simulink library "Parts_Lib"  (R2024a)
settings: Solver=ode45  StartTime=0.0  StopTime=10.0  RelTol=1e-3  EnableMultiTasking=on
undefined symbols (not defined in the file or in its folder): Extr_Data_Ring, X, Y, Z
libraries: sm_lib x44
(part 1 of 2)
Description:
  | Copyright 2015-2024 The MathWorks, Inc.
settings Model: Creator=smiller  LastModifiedBy=smiller
settings SolverCC: AlgebraicLoopSolver=TrustRegion
settings DataIOCC: LimitDataPoints=on  SaveFormat=Array  ReturnWorkspaceOutputs=off
settings OptimizationCC: ReuseModelBlockBuffer=off  LifeSpan=inf
settings DebuggingCC: SolverPrmCheckMsg=warning  UnconnectedInputMsg=warning  UnconnectedOutputMsg=warning  UnconnectedLineMsg=warning  AllowSymbolicDim=off  PregeneratedLibrarySubsystemCodeDiagnostic=none  SFUnexpectedBacktrackingDiag=warning  SFNoUnconditionalDefaultTransitionDiag=warning  SFExecutionAtInitializationDiag=none  ArithmeticOperatorsInVariantConditions=warning
settings HardwareCC: ProdBitPerPointer=32  ProdBitPerSizeT=32  ProdBitPerPtrDiffT=32  ProdLargestAtomicFloat=None  ProdIntDivRoundTo=Undefined  ProdEndianess=Unspecified  ProdWordSize=32  ProdHWDeviceType=32-bit Generic
settings ModelReferenceCC: EnableRefExpFcnMdlSchedulingChecks=on  PropagateSignalLabelsOutOfModel=off
settings SFSimCC: SimUseLocalCustomCode=off  CustomCodeUndefinedFunction=UseInterfaceOnly
settings RTWCC: RTWUseLocalCustomCode=off  GPUComputeCapability=3.5  DLArmComputeVersion=19.05
settings CodeAppCC: StateflowObjectComments=on
settings GRTTargetCC: TargetLangStandard=C89/C90 (ANSI)
settings ConfigComp: CovMetricSettings=dw  CovSaveCumulativeToWorkspaceVar=on  CovSaveSingleToWorkspaceVar=on  CovExternalEMLEnable=off  CovSFcnEnable=off

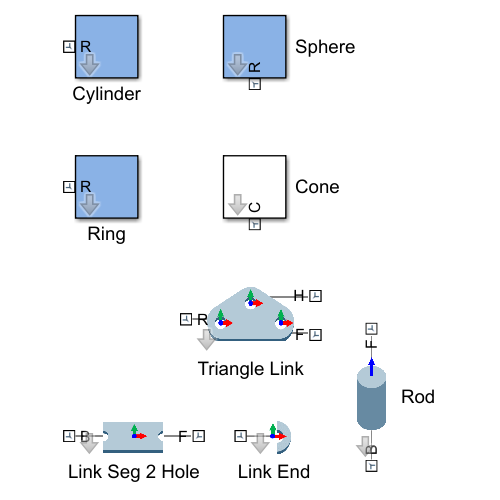
[thumbnail: Simulink's stored preview of the top-level diagram]
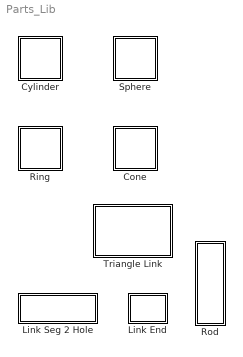
== system Parts_Lib ==
  Cone : Subsystem  mask(Conical Frustrum){cone_or=37.5e-3, cone_ir=30e-3, cone_h=4e-2, cone_theta=60, cone_angle_range=[-180 180], cone_rho=7000, cone_clr=[0.0 0.4 0.6], cone_opc=1, popup_markings=Two, mark_radius_scale=[1.01 1.01], mark_angle_range=2, mark_color=[1 1 1]}
      mask prompts: cone_or "Outer Radius (m):"; cone_ir "Inner Radius (m):"; cone_h "Height (m):"; cone_theta "Angle (deg):"; cone_angle_range "Sweep Angle (min, max angle (deg))"; cone_rho "Density (kg/m^3):"; cone_clr "Color [RGB]:"; cone_opc "Opacity (0-1)"; popup_markings "Show Markings"; mark_radius_scale "Radius scale factor [rad, h] (~1)"; mark_angle_range "Sweep Angle [0-180] (deg)"; mark_color "Color [RGB]"
      mask help:
      | This block models a conical frustrum.
      |
      | The port C corresponds to the frame at one end of the cone whose z-axis points along the cone axis.
      mask init:
      | frcon_xsec = Extr_Data_Frustum_Conical(cone_or, cone_theta, cone_h, cone_ir);
      | mark_xsec = Extr_Data_Frustum_Conical(cone_or*mark_radius_scale(1), cone_theta, cone_h*(1+(mark_radius_scale(2)-1)*2), cone_ir*(2-mark_radius_scale(1)));
      | 
      | mark_xsec(:,2) = mark_xsec(:,2)-cone_h*(mark_radius_scale(2)-1);
      | 
      | mark_1_opc = 0;
      | mark_2_opc = 0;
      | 
      | if(popup_markings == 2)
      |     mark_1_opc = 1;
      | elseif(popup_markings == 3)
      |     mark_1_opc = 1;
      |     mark_2_opc = 1;
      | end
      mask TypeOptions popup_markings: None | One | Two
      mask Callback popup_markings:
      | maskObj = Simulink.Mask.get(gcb);
      | mkc_h = maskObj.getDialogControl('container_markings');
      | if strcmp(get_param(gcb,'popup_markings'),'None')
      |     mkc_h.Visible = 'off';
      | else
      |     mkc_h.Visible = 'on';
      | end
      | clear maskObj mkc_h
      mask DialogControl Control2 Prompt: Plot Profile
      mask DialogControl Control2 Callback:
      | v = get_param(gcb,'MaskWSVariables');
      | getMaskValue = containers.Map({v.Name}',{v.Value}');
      | evalin('base',...
      |     sprintf('Extr_Data_Frustum_Conical(%s,%s,%s,%s,''%s'');',...
      |     num2str(getMaskValue('cone_or')),...
      |     num2str(getMaskValue('cone_theta')),...
      |     num2str(getMaskValue('cone_h')),...
      |     num2str(getMaskValue('cone_ir')),'plot'));
  Cylinder : Subsystem  Tag=CustomStyle  mask(Solid Cylinder with Markings){cyl_radius=0.5, cyl_length=0.2, cyl_density=1000, cyl_color=blue, cyl_opacity=1, cyl_color_custom=[0.7920    0.9900    0.9900], mark_radius=[0.75 0.5], mark_len_factor=1.01, mark_angle=60, mark_color=purple, mark_opacity=1}
      mask prompts: cyl_radius "Radius (m)"; cyl_length "Length (m)"; cyl_density "Density (kg/m^3)"; cyl_color "Color"; cyl_opacity "Opacity (0-1)"; cyl_color_custom "Custom Color (rgb)"; mark_radius "Outer, inner radius (% of cylinder radius)"; mark_len_factor "Length (factor of cylinder length)"; mark_angle "Sweep angle (deg)"; mark_color "Color"; mark_opacity "Opacity (0-1)"
      mask init:
      | curblk = gcb;
      | if strcmp(get_param(curblk,'cyl_color'),'red')
      |     set_param([curblk '/Cylinder'],'GraphicDiffuseColor','[0.8 0.0 0.2]');
      |     set_param(curblk,'BackGroundColor','[0.901961, 0.396078, 0.396078]');
      | elseif strcmp(get_param(gcb,'cyl_color'),'blue')
      |     set_param([curblk '/Cylinder'],'GraphicDiffuseColor','[0.0 0.5 0.7]');
      |     set_param(curblk,'BackGroundColor','[0.541176, 0.698039, 0.901961]');
      | elseif strcmp(get_param(gcb,'cyl_color'),'yellow')
      |     set_param([curblk '/Cylinder'],'GraphicDiffuseColor','[1.0 1.0 0.0]');
      |     set_param(curblk,'BackGroundColor','[0.905882, 0.890196, 0.392157]');
      | elseif strcmp(get_param(gcb,'cyl_color'),'gray')
      |     set_param([curblk '/Cylinder'],'GraphicDiffuseColor','[1.0 1.0 1.0]*0.6');
      |     set_param(curblk,'BackGroundColor','[0.6 0.6 0.6]');
      | elseif strcmp(get_param(gcb,'cyl_color'),'custom')
      |     set_param([curblk '/Cylinder'],'GraphicDiffuseColor',get_param(curblk,'cyl_color_custom'));
      |     set_param(curblk,'BackGroundColor','[1 1 1]');
      | end
      | 
      | if strcmp(get_param(curblk,'mark_color'),'purple')
      |     set_param([curblk '/Vis1'],'GraphicDiffuseColor','[0.4 0.0 0.4]');
      |     set_param([curblk '/Vis2'],'GraphicDiffuseColor','[0.4 0.0 0.4]');
      | elseif strcmp(get_param(gcb,'mark_color'),'green')
      |     set_param([curblk '/Vis1'],'GraphicDiffuseColor','[0.0 0.8 0.0]');
      |     set_param([curblk '/Vis2'],'GraphicDiffuseColor','[0.0 0.8 0.0]');
      | elseif strcmp(get_param(gcb,'mark_color'),'orange')
      |     set_param([curblk '/Vis1'],'GraphicDiffuseColor','[1.0 0.6 0.0]');
      |     set_param([curblk '/Vis2'],'GraphicDiffuseColor','[1.0 0.6 0.0]');
      | elseif strcmp(get_param(gcb,'mark_color'),'black')
      |     set_param([curblk '/Vis1'],'GraphicDiffuseColor','[0.0 0.0 0.0]');
      |     set_param([curblk '/Vis2'],'GraphicDiffuseColor','[0.0 0.0 0.0]');
      | end
      | 
      | clear curblk
      mask TypeOptions cyl_color: red | gray | yellow | blue | custom
      mask Callback cyl_color:
      | maskObj = Simulink.Mask.get(gcb);
      | clr_h = maskObj.getParameter('cyl_color_custom');
      | if strcmp(get_param(gcb,'cyl_color'),'custom')
      |     clr_h.Visible = 'on';
      | else
      |     clr_h.Visible = 'off';
      | end
      mask TypeOptions mark_color: purple | green | orange | black
      mask DialogControl Container4 Prompt: Cylinder
      mask DialogControl Container7 Prompt: Markings
  Link End : Subsystem  mask(Link End){circ_radout=0.025/2, circ_radin=0.005, popup_holelr=+X, deg_1=-90, deg_2=90, circ_len=0.01, circ_rho=7000, circ_color=[0 0.4 0.6], circ_opc=1}
      mask prompts: circ_radout "Outer Radius (m)"; circ_radin "Hole Radius (m)"; popup_holelr "Hole Side"; deg_1 "Start Angle (deg)"; deg_2 "Finish Angle (deg)"; circ_len "Thickness (m)"; circ_rho "Density (kg/m^3)"; circ_color "Color [RGB]"; circ_opc "Opacity (0-1)"
      mask help: Round end of Link. Define outer radius, hole radius, and hole placement. Port is at the hole center.
      mask init:
      | if(strcmpi(get_param(gcb,'popup_holelr'),'+X'));
      |     set_param(gcb,'deg_1','-90','deg_2','90');
      | else
      |     set_param(gcb,'deg_1','90','deg_2','270');
      | end
      | circ_xsec = Extr_Data_Ring(circ_radout, circ_radin, deg_1, deg_2);
      mask TypeOptions popup_holelr: -X | +X
      mask DialogControl Control12 Prompt: Plot Profile
      mask DialogControl Control12 Callback:
      | v = get_param(gcb,'MaskWSVariables');
      | getMaskValue = containers.Map({v.Name}',{v.Value}');
      | 
      | if(strcmp(get_param(gcb,'popup_holelr'),'+X'))
      |     evalin('base',...
      |         sprintf('Extr_Data_Ring(%s,%s,%s,%s,''%s'');',...
      |         num2str(getMaskValue('circ_radout')),...
      |         num2str(getMaskValue('circ_radin')),...
      |         '-90',...
      |         '90','plot'));
      | else
      |     evalin('base',...
      |         sprintf('Extr_Data_Ring(%s,%s,%s,%s,''%s'');',...
      |         num2str(getMaskValue('circ_radout')),...
      |         num2str(getMaskValue('circ_radin')),...
      |         '90',...
      |         '270','plot'));
      | end
      mask Display:
      | if(strcmp(get_param(gcb,'popup_holelr'),'+X'))
      |     image('Link_End_px_IMAGE.png');
      | else
      |     image('Link_End_nx_IMAGE.png');
      | end
  Link Seg 2 Hole : Subsystem  mask(Link Segment with 2 Holes){link_len=0.05, link_width=0.025, link_radh=0.005, link_thickness=0.01, link_rho=7000, link_color=[0 0.4 0.6], link_opc=1}
      mask prompts: link_len "Length (m)"; link_width "Width (m)"; link_radh "Hole Radius (m)"; link_thickness "Thickness (m)"; link_rho "Density (kg/m^3)"; link_color "Color [RGB]"; link_opc "Opacity (0-1)"
      mask help: Link segment with one hole. Define outer dimensions and hole radius. The interface ports are at either end of the link segment.
      mask init:
      | link_xsec = Extr_Data_Link2Hole(link_len, link_width, link_radh);
      mask DialogControl Control12 Prompt: Plot Profile
      mask DialogControl Control12 Callback:
      | v = get_param(gcb,'MaskWSVariables');
      | getMaskValue = containers.Map({v.Name}',{v.Value}');
      | evalin('base',...
      |     sprintf('Extr_Data_Link2Hole(%s,%s,%s,''%s'');',...
      |     num2str(getMaskValue('link_len')),...
      |     num2str(getMaskValue('link_width')),...
      |     num2str(getMaskValue('link_radh')),'plot'));
      mask Display: image('Link_Seg_2_Hole_IMAGE.png');
  Ring : Subsystem  Tag=CustomStyle  mask(Solid Cylinder with Markings){outer_rad=0.5, inner_rad=0.4, ring_length=0.2, ring_swpang=[0 360], ring_density=1000, ring_color=blue, ring_opacity=1, mark_radius=[0.95 1.05], mark_angle=60, mark_color=purple, mark_opacity=1}
      mask prompts: outer_rad "Outer Radius (m)"; inner_rad "Inner Radius (m)"; ring_length "Length (m)"; ring_swpang "Sweep Angles (deg)"; ring_density "Density (kg/m^3)"; ring_color "Color"; ring_opacity "Opacity (0-1)"; mark_radius "Outer, inner radius (% of outer, inner radius)"; mark_angle "Sweep angle (deg)"; mark_color "Color"; mark_opacity "Opacity (0-1)"
      mask init:
      | curblk = gcb;
      | if strcmp(get_param(curblk,'ring_color'),'red')
      |     set_param([curblk '/Ring'],'GraphicDiffuseColor','[0.8 0.0 0.2]');
      |     set_param(curblk,'BackGroundColor','[0.901961, 0.396078, 0.396078]');
      | elseif strcmp(get_param(gcb,'ring_color'),'blue')
      |     set_param([curblk '/Ring'],'GraphicDiffuseColor','[0.0 0.5 0.7]');
      |     set_param(curblk,'BackGroundColor','[0.541176, 0.698039, 0.901961]');
      | elseif strcmp(get_param(gcb,'ring_color'),'yellow')
      |     set_param([curblk '/Ring'],'GraphicDiffuseColor','[1.0 1.0 0.0]');
      |     set_param(curblk,'BackGroundColor','[0.905882, 0.890196, 0.392157]');
      | elseif strcmp(get_param(gcb,'ring_color'),'gray')
      |     set_param([curblk '/Ring'],'GraphicDiffuseColor','[0.5 0.5 0.5]');
      |     set_param(curblk,'BackGroundColor','[0.796078, 0.796078, 0.796078]');
      | end
      | 
      | if strcmp(get_param(curblk,'mark_color'),'purple')
      |     set_param([curblk '/Vis1'],'GraphicDiffuseColor','[0.4 0.0 0.4]');
      |     set_param([curblk '/Vis2'],'GraphicDiffuseColor','[0.4 0.0 0.4]');
      | elseif strcmp(get_param(gcb,'mark_color'),'green')
      |     set_param([curblk '/Vis1'],'GraphicDiffuseColor','[0.0 0.8 0.0]');
      |     set_param([curblk '/Vis2'],'GraphicDiffuseColor','[0.0 0.8 0.0]');
      | elseif strcmp(get_param(gcb,'mark_color'),'orange')
      |     set_param([curblk '/Vis1'],'GraphicDiffuseColor','[1.0 0.6 0.0]');
      |     set_param([curblk '/Vis2'],'GraphicDiffuseColor','[1.0 0.6 0.0]');
      | elseif strcmp(get_param(gcb,'mark_color'),'black')
      |     set_param([curblk '/Vis1'],'GraphicDiffuseColor','[0.0 0.0 0.0]');
      |     set_param([curblk '/Vis2'],'GraphicDiffuseColor','[0.0 0.0 0.0]');
      | end
      | 
      | clear curblk
      mask TypeOptions ring_color: red | gray | yellow | blue
      mask TypeOptions mark_color: purple | green | orange | black
      mask DialogControl Container4 Prompt: Ring
      mask DialogControl Container7 Prompt: Markings
  Rod : Subsystem  mask(Rod){rod_rad=0.005, rod_len=0.0125, rod_rho=7000, rod_color=[0.5 0.5 0.5], popup_zori=Local +Z, popup_markings=None, mark_radius_range=[0.5 1.01], mark_length_range=1.005, mark_angle_range=30, mark_color=[1 1 1]}
      mask prompts: rod_rad "Radius (m)"; rod_len "Length (m)"; rod_rho "Density (kg/m^3)"; rod_color "Color [RGB]"; popup_zori "Relative Position (B to F)"; popup_markings "Show Markings"; mark_radius_range "Radial Range [min max] (0-1.1)"; mark_length_range "Length Range (0-1.1)"; mark_angle_range "Sweep Angle [0-180] (deg)"; mark_color "Color [RGB]"
      mask help:
      | This block models a rod.
      |
      | The two interface ports corresponds to the frames at either end of the rod which are along the z-axis.
      mask init:
      | mark_xsec =  [
      |     rod_rad*max(mark_radius_range) rod_len*mark_length_range/2; 
      |     rod_rad*min(mark_radius_range) rod_len*mark_length_range/2; 
      |     rod_rad*min(mark_radius_range) -rod_len*mark_length_range/2; 
      |     rod_rad*max(mark_radius_range) -rod_len*mark_length_range/2];
      | 
      | mark_1_opc = 0;
      | mark_2_opc = 0;
      | 
      | if(popup_markings == 2)
      |     mark_1_opc = 1;
      | elseif(popup_markings == 3)
      |     mark_1_opc = 1;
      |     mark_2_opc = 1;
      | end
      | 
      | if(popup_zori == 2)
      |     z_ori = -1;
      | else
      |     z_ori = 1;
      | end
      mask TypeOptions popup_zori: Local +Z | Local -Z
      mask TypeOptions popup_markings: None | One | Two
      mask Callback popup_markings:
      | maskObj = Simulink.Mask.get(gcb);
      | mkc_h = maskObj.getDialogControl('container_markings');
      | if strcmp(get_param(gcb,'popup_markings'),'None')
      |     mkc_h.Visible = 'off';
      | else
      |     mkc_h.Visible = 'on';
      | end
      | clear maskObj mkc_h
      mask Display:
      | if(popup_zori == 2)
      |     image('Rod_nZ_IMAGE.png')
      | else
      |     image('Rod_pZ_IMAGE.png')
      | end
  Sphere : Subsystem  Tag=CustomStyle  mask(Sphere with Markings){sph_radius=0.01, sph_density=1000, sph_color=blue, sph_opacity=1, mark_type=Arcs about axes, arc_width=[40 50], arc_angle=60, ring_width=5, ring_irad=0.95, mark_color=black, mark_opacity_x=1, mark_opacity_y=1, mark_opacity_z=1, mark_opacity=1, ring_opacity=0, arc_opacity=0, arc_extr_data=0}
      mask prompts: sph_radius "Radius (m)"; sph_density "Density (kg/m^3)"; sph_color "Color"; sph_opacity "Opacity"; mark_type "Marking Type"; arc_width "Arc width (start, end) (deg)"; arc_angle "Sweep angle (deg)"; ring_width "Ring Width (deg)"; ring_irad "Ring Inner Radius (% sphere radius)"; mark_color "Color"; mark_opacity_x "Opacity (0-1): X-Axis"; mark_opacity_y "Y-Axis"; mark_opacity_z "Z-Axis"; mark_opacity "Opacity"; ring_opacity "Ring Opacity"; arc_opacity "Arc Opacity"; arc_extr_data "Arc Extrusion Data (xy)"
      mask init:
      | curblk = gcb;
      | if strcmp(get_param(curblk,'sph_color'),'red')
      |     set_param([curblk '/Sphere'],'GraphicDiffuseColor','[0.8 0.0 0.2]');
      |     set_param(curblk,'BackGroundColor','[0.901961, 0.396078, 0.396078]');
      | elseif strcmp(get_param(gcb,'sph_color'),'blue')
      |     set_param([curblk '/Sphere'],'GraphicDiffuseColor','[0.0 0.5 0.7]');
      |     set_param(curblk,'BackGroundColor','[0.541176, 0.698039, 0.901961]');
      | elseif strcmp(get_param(gcb,'sph_color'),'yellow')
      |     set_param([curblk '/Sphere'],'GraphicDiffuseColor','[1.0 1.0 0.0]');
      |     set_param(curblk,'BackGroundColor','[0.905882, 0.890196, 0.392157]');
      | elseif strcmp(get_param(gcb,'sph_color'),'gray')
      |     set_param([curblk '/Sphere'],'GraphicDiffuseColor','[0.5 0.5 0.5]');
      |     set_param(curblk,'BackGroundColor','[0.796078, 0.796078, 0.796078]');
      | elseif strcmp(get_param(gcb,'sph_color'),'white')
      |     set_param([curblk '/Sphere'],'GraphicDiffuseColor','[1.0 1.0 1.0]');
      |     set_param(curblk,'BackGroundColor','[1, 1, 1]');
      | end
      | 
      | if strcmp(get_param(curblk,'mark_color'),'purple'), tmkclr = '[0.4 0.0 0.4]';
      | elseif strcmp(get_param(gcb,'mark_color'),'green'), tmkclr = '[0.0 0.8 0.0]';
      | elseif strcmp(get_param(gcb,'mark_color'),'orange'), tmkclr = '[1.0 0.6 0.0]';
      | elseif strcmp(get_param(gcb,'mark_color'),'black'), tmkclr = '[0.0 0.0 0.0]';
      | end
      | 
      | if strcmp(get_param(curblk,'mark_color'),'axes'),
      |     set_param([curblk '/Arcs/ArcZ1'],'GraphicDiffuseColor','[0.0 0.0 1.0]');
      |     set_param([curblk '/Arcs/ArcZ2'],'GraphicDiffuseColor','[0.0 0.0 1.0]');
      |     set_param([curblk '/Rings/RingZ'],'GraphicDiffuseColor','[0.0 0.0 1.0]');
      |     set_param([curblk '/Arcs/ArcY1'],'GraphicDiffuseColor','[0.0 1.0 0.0]');
      |     set_param([curblk '/Arcs/ArcY2'],'GraphicDiffuseColor','[0.0 1.0 0.0]');
      |     set_param([curblk '/Rings/RingY'],'GraphicDiffuseColor','[0.0 1.0 0.0]');
      |     set_param([curblk '/Arcs/ArcX1'],'GraphicDiffuseColor','[1.0 0.0 0.0]');
      |     set_param([curblk '/Arcs/ArcX2'],'GraphicDiffuseColor','[1.0 0.0 0.0]');
      |     set_param([curblk '/Rings/RingX'],'GraphicDiffuseColor','[1.0 0.0 0.0]');
      | else
      |     set_param([curblk '/Arcs/ArcZ1'],'GraphicDiffuseColor',tmkclr);
      |     set_param([curblk '/Arcs/ArcZ2'],'GraphicDiffuseColor',tmkclr);
      |     set_param([curblk '/Arcs/ArcY1'],'GraphicDiffuseColor',tmkclr);
      |     set_param([curblk '/Arcs/ArcY2'],'GraphicDiffuseColor',tmkclr);
      |     set_param([curblk '/Arcs/ArcX1'],'GraphicDiffuseColor',tmkclr);
      |     set_param([curblk '/Arcs/ArcX2'],'GraphicDiffuseColor',tmkclr);
      |     set_param([curblk '/Rings/RingX'],'GraphicDiffuseColor',tmkclr);
      |     set_param([curblk '/Rings/RingY'],'GraphicDiffuseColor',tmkclr);
      |     set_param([curblk '/Rings/RingZ'],'GraphicDiffuseColor',tmkclr);
      | end
      | 
      | arc_opacity = 0;
      | ring_opacity = 0;
      | 
      | if strcmp(get_param(curblk,'mark_type'),'Arcs about axes')
      |     arc_opacity = 1;
      | elseif strcmp(get_param(curblk,'mark_type'),'Rings on center planes')
      |     ring_opacity = 1;
      | end
      | 
      | %arc_extr_data = sph_radius*1.0001*[cosd(max(arc_width(2)):-(arc_width(2)-arc_width(1))/20:arc_width(1)) cosd(-arc_width(1):-(arc_width(2)-arc_width(1))/20:-arc_width(2));     sind(arc_width(2):-(arc_width(2)-arc_width(1))/20:arc_width(1)) sind(-arc_width(1):-(arc_width(2)-arc_width(1))/20:-arc_width(2))]';
      | arc_extr_data = sph_radius*1.0001*[cosd(min(arc_width):(max(arc_width)-min(arc_width))/20:max(arc_width)) cosd(-max(arc_width):(max(arc_width)-min(arc_width))/20:-min(arc_width)); sind(min(arc_width):(max(arc_width)-min(arc_width))/20:max(arc_width)) sind(-max(arc_width):(max(arc_width)-min(arc_width))/20:-min(arc_width))]';
      | clear curblk tmkclr
      mask TypeOptions sph_color: red | gray | yellow | blue | white
      mask TypeOptions mark_type: None | Arcs about axes | Rings on center planes
      mask Callback mark_type:
      | maskObj = Simulink.Mask.get(gcb);
      | arw_h = maskObj.getParameter('arc_width');
      | ara_h = maskObj.getParameter('arc_angle');
      | riw_h = maskObj.getParameter('ring_width');
      | rii_h = maskObj.getParameter('ring_irad');
      | mkc_h = maskObj.getParameter('mark_color');
      |     arw_h.Visible = 'off';
      |     ara_h.Visible = 'off';
      |     riw_h.Visible = 'off';
      |     rii_h.Visible = 'off';
      |     mkc_h.Visible = 'off';
      | if strcmp(get_param(gcb,'mark_type'),'Arcs about axes')
      |     arw_h.Visible = 'on';
      |     ara_h.Visible = 'on';
      |     mkc_h.Visible = 'on';
      | elseif strcmp(get_param(gcb,'mark_type'),'Rings on center planes')
      |     riw_h.Visible = 'on';
      |     rii_h.Visible = 'on';
      |     mkc_h.Visible = 'on';
      | end
      | clear maskObj
      mask TypeOptions mark_color: purple | green | orange | black | axes
      mask DialogControl Container4 Prompt: Sphere
      mask DialogControl Container7 Prompt: Markings
  Triangle Link : Subsystem  mask(Triangular Link with Rounded Corners){link_len=0.1, link_height=0.05, link_xlen=0.33, link_radh=0.005, link_rado=0.0125, link_thickness=0.01, link_rho=7000, link_color=[0 0.4 0.6], link_opc=1}
      mask prompts: link_len "Length (m)"; link_height "Height (m)"; link_xlen "Center Hole Position (0-1)"; link_radh "Hole Radius (m)"; link_rado "Link Outer Radius (m)"; link_thickness "Thickness (m)"; link_rho "Density (kg/m^3)"; link_color "Color [RGB]"; link_opc "Opacity (0-1)"
      mask help: Triangular link with rounded ends and 3 holes. Define outer dimensions, hole radius, and number of holes. The interface frames are at the center of each of the three holes.
      mask init:
      | link_xsec = Extr_Data_TriangleRounded_Holes(link_len, link_height, link_xlen, link_radh, link_rado);
      mask DialogControl Control12 Prompt: Plot Profile
      mask DialogControl Control12 Callback:
      | v = get_param(gcb,'MaskWSVariables');
      | getMaskValue = containers.Map({v.Name}',{v.Value}');
      | evalin('base',...
      |     sprintf('Extr_Data_TriangleRounded_Holes(%s,%s,%s,%s,%s,''%s'');',...
      |     num2str(getMaskValue('link_len')),...
      |     num2str(getMaskValue('link_height')),...
      |     num2str(getMaskValue('link_xlen')),...
      |     num2str(getMaskValue('link_radh')),...
      |     num2str(getMaskValue('link_rado')),'plot'));
      mask Display: image('Triangle_Link_IMAGE.png')

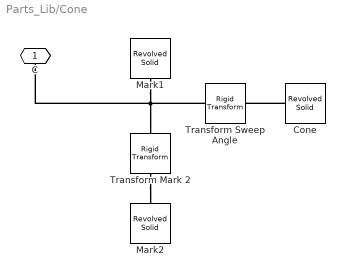
== system Parts_Lib/Cone ==
  Cone : sm_lib/Body Elements/Revolved Solid  RevolutionCrossSection=frcon_xsec  RevolutionCrossSectionUnits=m  RevolutionExtent=Custom  RevolutionAngle=cone_angle_range(2)-cone_angle_range(1)  RevolutionAngleUnits=deg  ExportConvexHullGeometry=off  InertiaType=CalculateFromGeometry  BasedOnType=Density  Density=cone_rho  DensityUnits=kg/(m^3)  Mass=1  MassUnits=kg  CenterOfMass=[0 0 0]  CenterOfMassUnits=m  MomentsOfInertia=[1 1 1]  MomentsOfInertiaUnits=kg*m^2  ProductsOfInertia=[0 0 0]  ProductsOfInertiaUnits=kg*m^2  GraphicType=FromGeometry  MarkerShape=Sphere  MarkerSize=10  GraphicVisPropType=SimpleVisualProperties  GraphicDiffuseColor=cone_clr  GraphicOpacity=cone_opc  GraphicSpecularColor=[0.5 0.5 0.5 1.0]  GraphicAmbientColor=[0.15 0.15 0.15 1.0]  GraphicEmissiveColor=[0.0 0.0 0.0 1.0]  GraphicShininess=75  DoExposeReferenceFrame=on  SerializedFrames=<Frames/>
  Mark1 : sm_lib/Body Elements/Revolved Solid  RevolutionCrossSection=mark_xsec  RevolutionCrossSectionUnits=m  RevolutionExtent=Custom  RevolutionAngle=mark_angle_range  RevolutionAngleUnits=deg  ExportConvexHullGeometry=off  InertiaType=CalculateFromGeometry  BasedOnType=Density  Density=0  DensityUnits=kg/m^3  Mass=1  MassUnits=kg  CenterOfMass=[0 0 0]  CenterOfMassUnits=m  MomentsOfInertia=[1 1 1]  MomentsOfInertiaUnits=kg*m^2  ProductsOfInertia=[1 1 1]  ProductsOfInertiaUnits=kg*m^2  GraphicType=FromGeometry  MarkerShape=Sphere  MarkerSize=10  GraphicVisPropType=SimpleVisualProperties  GraphicDiffuseColor=mark_color  GraphicOpacity=mark_1_opc  GraphicSpecularColor=[0.5 0.5 0.5 1.0]  GraphicAmbientColor=[0.15 0.15 0.15 1.0]  GraphicEmissiveColor=[0.0 0.0 0.0 1.0]  GraphicShininess=75  DoExposeReferenceFrame=on  SerializedFrames=<Frames/>
  Mark2 : sm_lib/Body Elements/Revolved Solid  RevolutionCrossSection=mark_xsec  RevolutionCrossSectionUnits=m  RevolutionExtent=Custom  RevolutionAngle=mark_angle_range  RevolutionAngleUnits=deg  ExportConvexHullGeometry=off  InertiaType=CalculateFromGeometry  BasedOnType=Density  Density=0  DensityUnits=kg/m^3  Mass=1  MassUnits=kg  CenterOfMass=[0 0 0]  CenterOfMassUnits=m  MomentsOfInertia=[1 1 1]  MomentsOfInertiaUnits=kg*m^2  ProductsOfInertia=[1 1 1]  ProductsOfInertiaUnits=kg*m^2  GraphicType=FromGeometry  MarkerShape=Sphere  MarkerSize=10  GraphicVisPropType=SimpleVisualProperties  GraphicDiffuseColor=mark_color  GraphicOpacity=mark_2_opc  GraphicSpecularColor=[0.5 0.5 0.5 1.0]  GraphicAmbientColor=[0.15 0.15 0.15 1.0]  GraphicEmissiveColor=[0.0 0.0 0.0 1.0]  GraphicShininess=75  DoExposeReferenceFrame=on  SerializedFrames=<Frames/>
  Transform Mark 2 : sm_lib/Frames and Transforms/Rigid Transform  RotationMethod=StandardAxis  FollAlignAxisA=+X  BaseAlignAxisA=+Y  FollAlignAxisB=+Y  BaseAlignAxisB=+Z  RotationStandardAxis=+Z  RotationAngle=180  RotationAngleUnits=deg  RotationArbitraryAxis=[0 0 1]  RotationSequenceAxes=FollowerAxes  RotationSequence=XYX  RotationSequenceAngles=[0 0 0]  RotationSequenceAnglesUnits=deg  RotationMatrix=[1 0 0; 0 1 0; 0 0 1]  Quaternion=[1 0 0 0]  TranslationMethod=None  TranslationCartesianOffset=[0 0 0]  TranslationCartesianOffsetUnits=m  TranslationStandardAxis=+Z  TranslationStandardOffset=0  TranslationStandardOffsetUnits=m  TranslationROffset=0  TranslationROffsetUnits=m  TranslationThetaOffset=0  TranslationThetaOffsetUnits=deg  TranslationZOffset=0  TranslationZOffsetUnits=m
  Transform Sweep Angle : sm_lib/Frames and Transforms/Rigid Transform  RotationMethod=StandardAxis  FollAlignAxisA=+X  BaseAlignAxisA=+Y  FollAlignAxisB=+Y  BaseAlignAxisB=+Z  RotationStandardAxis=+Z  RotationAngle=(cone_angle_range(2)+cone_angle_range(1))/2  RotationAngleUnits=deg  RotationArbitraryAxis=[0 0 1]  RotationSequenceAxes=FollowerAxes  RotationSequence=XYX  RotationSequenceAngles=[0 0 0]  RotationSequenceAnglesUnits=deg  RotationMatrix=[1 0 0; 0 1 0; 0 0 1]  Quaternion=[1 0 0 0]  TranslationMethod=None  TranslationCartesianOffset=[0 0 0]  TranslationCartesianOffsetUnits=m  TranslationStandardAxis=+Z  TranslationStandardOffset=0  TranslationStandardOffsetUnits=m  TranslationROffset=0  TranslationROffsetUnits=m  TranslationThetaOffset=0  TranslationThetaOffsetUnits=deg  TranslationZOffset=0  TranslationZOffsetUnits=m
  C : PMIOPort  Side=Right
  connections:
  Cone/RConn1 -- Transform Sweep Angle/RConn1
  Transform Mark 2/RConn1 -- Mark2/RConn1
  Mark1/RConn1 -- C/RConn1 -- Transform Sweep Angle/LConn1 -- Transform Mark 2/LConn1

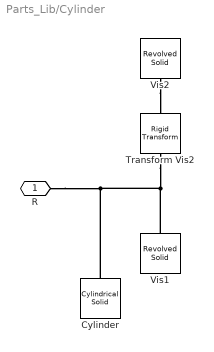
== system Parts_Lib/Cylinder ==
  Cylinder : sm_lib/Body Elements/Cylindrical Solid  CylinderRadius=cyl_radius  CylinderRadiusUnits=m  CylinderLength=cyl_length  CylinderLengthUnits=m  ExportEntireGeometry=off  InertiaType=CalculateFromGeometry  BasedOnType=Density  Density=cyl_density  DensityUnits=kg/(m^3)  Mass=1  MassUnits=kg  CenterOfMass=[0 0 0]  CenterOfMassUnits=m  MomentsOfInertia=[1 1 1]  MomentsOfInertiaUnits=kg*m^2  ProductsOfInertia=[0 0 0]  ProductsOfInertiaUnits=kg*m^2  GraphicType=FromGeometry  MarkerShape=Sphere  MarkerSize=10  GraphicVisPropType=SimpleVisualProperties  GraphicDiffuseColor=[0.0 0.5 0.7]  GraphicOpacity=cyl_opacity  GraphicSpecularColor=[0.5 0.5 0.5 1.0]  GraphicAmbientColor=[0.15 0.15 0.15 1.0]  GraphicEmissiveColor=[0.0 0.0 0.0 1.0]  GraphicShininess=75  DoExposeReferenceFrame=on  SerializedFrames=<Frames/>
  Transform Vis2 : sm_lib/Frames and Transforms/Rigid Transform  RotationMethod=StandardAxis  FollAlignAxisA=+X  BaseAlignAxisA=+Y  FollAlignAxisB=+Y  BaseAlignAxisB=+Z  RotationStandardAxis=+Y  RotationAngle=180  RotationAngleUnits=deg  RotationArbitraryAxis=[0 0 1]  RotationSequenceAxes=FollowerAxes  RotationSequence=XYX  RotationSequenceAngles=[0 0 0]  RotationSequenceAnglesUnits=deg  RotationMatrix=[1 0 0; 0 1 0; 0 0 1]  Quaternion=[1 0 0 0]  TranslationMethod=None  TranslationCartesianOffset=[0 0 0]  TranslationCartesianOffsetUnits=m  TranslationStandardAxis=+Z  TranslationStandardOffset=0  TranslationStandardOffsetUnits=m  TranslationROffset=0  TranslationROffsetUnits=m  TranslationThetaOffset=0  TranslationThetaOffsetUnits=deg  TranslationZOffset=0  TranslationZOffsetUnits=m
  Vis1 : sm_lib/Body Elements/Revolved Solid  RevolutionCrossSection=[cyl_radius*mark_radius(1) cyl_length/2*mark_len_factor; cyl_radius*mark_radius(2) cyl_length/2*mark_len_factor; cyl_radius*mark_radius(2) -cyl_length/2*mark_len_factor; cyl_radius*mark_radius(1) -cyl_length/2*mark_len_factor]  RevolutionCrossSectionUnits=m  RevolutionExtent=Custom  RevolutionAngle=mark_angle  RevolutionAngleUnits=deg  ExportConvexHullGeometry=off  InertiaType=CalculateFromGeometry  BasedOnType=Density  Density=1e-3  DensityUnits=kg/(m^3)  Mass=1  MassUnits=kg  CenterOfMass=[0 0 0]  CenterOfMassUnits=m  MomentsOfInertia=[1 1 1]  MomentsOfInertiaUnits=kg*m^2  ProductsOfInertia=[0 0 0]  ProductsOfInertiaUnits=kg*m^2  GraphicType=FromGeometry  MarkerShape=Sphere  MarkerSize=10  GraphicVisPropType=SimpleVisualProperties  GraphicDiffuseColor=[0.4 0.0 0.4]  GraphicOpacity=mark_opacity  GraphicSpecularColor=[0.5 0.5 0.5 1.0]  GraphicAmbientColor=[0.15 0.15 0.15 1.0]  GraphicEmissiveColor=[0.0 0.0 0.0 1.0]  GraphicShininess=75  DoExposeReferenceFrame=on  SerializedFrames=<Frames/>
  Vis2 : sm_lib/Body Elements/Revolved Solid  RevolutionCrossSection=[cyl_radius*mark_radius(1) cyl_length/2*mark_len_factor; cyl_radius*mark_radius(2) cyl_length/2*mark_len_factor; cyl_radius*mark_radius(2) -cyl_length/2*mark_len_factor; cyl_radius*mark_radius(1) -cyl_length/2*mark_len_factor]  RevolutionCrossSectionUnits=m  RevolutionExtent=Custom  RevolutionAngle=mark_angle  RevolutionAngleUnits=deg  ExportConvexHullGeometry=off  InertiaType=CalculateFromGeometry  BasedOnType=Density  Density=1e-3  DensityUnits=kg/(m^3)  Mass=1  MassUnits=kg  CenterOfMass=[0 0 0]  CenterOfMassUnits=m  MomentsOfInertia=[1 1 1]  MomentsOfInertiaUnits=kg*m^2  ProductsOfInertia=[0 0 0]  ProductsOfInertiaUnits=kg*m^2  GraphicType=FromGeometry  MarkerShape=Sphere  MarkerSize=10  GraphicVisPropType=SimpleVisualProperties  GraphicDiffuseColor=[0.4 0.0 0.4]  GraphicOpacity=mark_opacity  GraphicSpecularColor=[0.5 0.5 0.5 1.0]  GraphicAmbientColor=[0.15 0.15 0.15 1.0]  GraphicEmissiveColor=[0.0 0.0 0.0 1.0]  GraphicShininess=75  DoExposeReferenceFrame=on  SerializedFrames=<Frames/>
  R : PMIOPort  Side=Left
  connections:
  Vis2/RConn1 -- Transform Vis2/RConn1
  Vis1/RConn1 -- Transform Vis2/LConn1 -- Cylinder/RConn1 -- R/RConn1

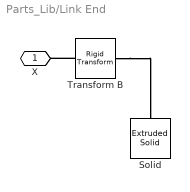
== system Parts_Lib/Link End ==
  Solid : sm_lib/Body Elements/Extruded Solid  ExtrusionType=General  PolygonNumSides=3  PolygonOuterRadius=1  PolygonOuterRadiusUnits=m  ExportEntireGeometry=off  ExtrusionCrossSection=circ_xsec  ExtrusionCrossSectionUnits=m  ExportConvexHullGeometry=off  ExtrusionLength=circ_len  ExtrusionLengthUnits=m  InertiaType=CalculateFromGeometry  BasedOnType=Density  Density=circ_rho  DensityUnits=kg/(m^3)  Mass=1  MassUnits=kg  CenterOfMass=[0 0 0]  CenterOfMassUnits=m  MomentsOfInertia=[1 1 1]  MomentsOfInertiaUnits=kg*m^2  ProductsOfInertia=[0 0 0]  ProductsOfInertiaUnits=kg*m^2  GraphicType=FromGeometry  MarkerShape=Sphere  MarkerSize=10  GraphicVisPropType=SimpleVisualProperties  GraphicDiffuseColor=circ_color  GraphicOpacity=circ_opc  GraphicSpecularColor=[0.5 0.5 0.5 1.0]  GraphicAmbientColor=[0.15 0.15 0.15 1.0]  GraphicEmissiveColor=[0.0 0.0 0.0 1.0]  GraphicShininess=75  DoExposeReferenceFrame=on  SerializedFrames=<Frames/>
  Transform B : sm_lib/Frames and Transforms/Rigid Transform  RotationMethod=StandardAxis  FollAlignAxisA=+X  BaseAlignAxisA=+Y  FollAlignAxisB=+Y  BaseAlignAxisB=+Z  RotationStandardAxis=+Y  RotationAngle=0  RotationAngleUnits=deg  RotationArbitraryAxis=[0 0 1]  RotationSequenceAxes=FollowerAxes  RotationSequence=XYX  RotationSequenceAngles=[0 0 0]  RotationSequenceAnglesUnits=deg  RotationMatrix=[1 0 0; 0 1 0; 0 0 1]  Quaternion=[1 0 0 0]  TranslationMethod=None  TranslationCartesianOffset=[0 0 0]  TranslationCartesianOffsetUnits=m  TranslationStandardAxis=+X  TranslationStandardOffset=0  TranslationStandardOffsetUnits=m  TranslationROffset=0  TranslationROffsetUnits=m  TranslationThetaOffset=0  TranslationThetaOffsetUnits=deg  TranslationZOffset=0  TranslationZOffsetUnits=m
  X : PMIOPort  Side=Left
  connections:
  Transform B/RConn1 -- Solid/RConn1
  Transform B/LConn1 -- X/RConn1

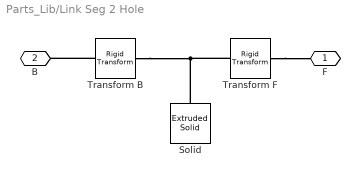
== system Parts_Lib/Link Seg 2 Hole ==
  Solid : sm_lib/Body Elements/Extruded Solid  ExtrusionType=General  PolygonNumSides=3  PolygonOuterRadius=1  PolygonOuterRadiusUnits=m  ExportEntireGeometry=off  ExtrusionCrossSection=link_xsec  ExtrusionCrossSectionUnits=m  ExportConvexHullGeometry=off  ExtrusionLength=link_thickness  ExtrusionLengthUnits=m  InertiaType=CalculateFromGeometry  BasedOnType=Density  Density=link_rho  DensityUnits=kg/(m^3)  Mass=1  MassUnits=kg  CenterOfMass=[0 0 0]  CenterOfMassUnits=m  MomentsOfInertia=[1 1 1]  MomentsOfInertiaUnits=kg*m^2  ProductsOfInertia=[0 0 0]  ProductsOfInertiaUnits=kg*m^2  GraphicType=FromGeometry  MarkerShape=Sphere  MarkerSize=10  GraphicVisPropType=SimpleVisualProperties  GraphicDiffuseColor=link_color  GraphicOpacity=link_opc  GraphicSpecularColor=[0.5 0.5 0.5 1.0]  GraphicAmbientColor=[0.15 0.15 0.15 1.0]  GraphicEmissiveColor=[0.0 0.0 0.0 1.0]  GraphicShininess=75  DoExposeReferenceFrame=on  SerializedFrames=<Frames/>
  Transform B : sm_lib/Frames and Transforms/Rigid Transform  RotationMethod=None  FollAlignAxisA=+X  BaseAlignAxisA=+Y  FollAlignAxisB=+Y  BaseAlignAxisB=+Z  RotationStandardAxis=+Z  RotationAngle=0.0  RotationAngleUnits=deg  RotationArbitraryAxis=[0 0 1]  RotationSequenceAxes=FollowerAxes  RotationSequence=XYX  RotationSequenceAngles=[0 0 0]  RotationSequenceAnglesUnits=deg  RotationMatrix=[1 0 0; 0 1 0; 0 0 1]  Quaternion=[1 0 0 0]  TranslationMethod=StandardAxis  TranslationCartesianOffset=[0 0 0]  TranslationCartesianOffsetUnits=m  TranslationStandardAxis=-X  TranslationStandardOffset=link_len/2  TranslationStandardOffsetUnits=m  TranslationROffset=0  TranslationROffsetUnits=m  TranslationThetaOffset=0  TranslationThetaOffsetUnits=deg  TranslationZOffset=0  TranslationZOffsetUnits=m
  Transform F : sm_lib/Frames and Transforms/Rigid Transform  RotationMethod=None  FollAlignAxisA=+X  BaseAlignAxisA=+Y  FollAlignAxisB=+Y  BaseAlignAxisB=+Z  RotationStandardAxis=+Z  RotationAngle=0.0  RotationAngleUnits=deg  RotationArbitraryAxis=[0 0 1]  RotationSequenceAxes=FollowerAxes  RotationSequence=XYX  RotationSequenceAngles=[0 0 0]  RotationSequenceAnglesUnits=deg  RotationMatrix=[1 0 0; 0 1 0; 0 0 1]  Quaternion=[1 0 0 0]  TranslationMethod=StandardAxis  TranslationCartesianOffset=[0 0 0]  TranslationCartesianOffsetUnits=m  TranslationStandardAxis=+X  TranslationStandardOffset=link_len/2  TranslationStandardOffsetUnits=m  TranslationROffset=0  TranslationROffsetUnits=m  TranslationThetaOffset=0  TranslationThetaOffsetUnits=deg  TranslationZOffset=0  TranslationZOffsetUnits=m
  F : PMIOPort  Side=Right
  B : PMIOPort  Port=2  Side=Left
  connections:
  Transform F/RConn1 -- F/RConn1
  Transform B/RConn1 -- B/RConn1
  Transform B/LConn1 -- Transform F/LConn1 -- Solid/RConn1

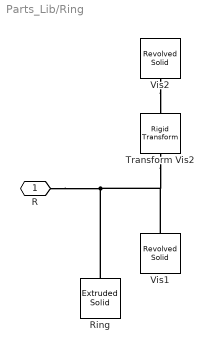
== system Parts_Lib/Ring ==
  Ring : sm_lib/Body Elements/Extruded Solid  ExtrusionType=General  PolygonNumSides=3  PolygonOuterRadius=1  PolygonOuterRadiusUnits=m  ExportEntireGeometry=off  ExtrusionCrossSection=Extr_Data_Ring(outer_rad,inner_rad,ring_swpang(1),ring_swpang(2))  ExtrusionCrossSectionUnits=m  ExportConvexHullGeometry=off  ExtrusionLength=ring_length  ExtrusionLengthUnits=m  InertiaType=CalculateFromGeometry  BasedOnType=Density  Density=ring_density  DensityUnits=kg/(m^3)  Mass=1  MassUnits=kg  CenterOfMass=[0 0 0]  CenterOfMassUnits=m  MomentsOfInertia=[1 1 1]  MomentsOfInertiaUnits=kg*m^2  ProductsOfInertia=[0 0 0]  ProductsOfInertiaUnits=kg*m^2  GraphicType=FromGeometry  MarkerShape=Sphere  MarkerSize=10  GraphicVisPropType=SimpleVisualProperties  GraphicDiffuseColor=[0.0 0.5 0.7]  GraphicOpacity=ring_opacity  GraphicSpecularColor=[0.5 0.5 0.5 1.0]  GraphicAmbientColor=[0.15 0.15 0.15 1.0]  GraphicEmissiveColor=[0.0 0.0 0.0 1.0]  GraphicShininess=75  DoExposeReferenceFrame=on  SerializedFrames=<Frames/>
  Transform Vis2 : sm_lib/Frames and Transforms/Rigid Transform  RotationMethod=StandardAxis  FollAlignAxisA=+X  BaseAlignAxisA=+Y  FollAlignAxisB=+Y  BaseAlignAxisB=+Z  RotationStandardAxis=+Y  RotationAngle=180  RotationAngleUnits=deg  RotationArbitraryAxis=[0 0 1]  RotationSequenceAxes=FollowerAxes  RotationSequence=XYX  RotationSequenceAngles=[0 0 0]  RotationSequenceAnglesUnits=deg  RotationMatrix=[1 0 0; 0 1 0; 0 0 1]  Quaternion=[1 0 0 0]  TranslationMethod=None  TranslationCartesianOffset=[0 0 0]  TranslationCartesianOffsetUnits=m  TranslationStandardAxis=+Z  TranslationStandardOffset=0  TranslationStandardOffsetUnits=m  TranslationROffset=0  TranslationROffsetUnits=m  TranslationThetaOffset=0  TranslationThetaOffsetUnits=deg  TranslationZOffset=0  TranslationZOffsetUnits=m
  Vis1 : sm_lib/Body Elements/Revolved Solid  RevolutionCrossSection=[outer_rad*mark_radius(1) ring_length/2*1.002; inner_rad*mark_radius(2) ring_length/2*1.002; inner_rad*mark_radius(2) -ring_length/2*1.002; outer_rad*mark_radius(1) -ring_length/2*1.002]  RevolutionCrossSectionUnits=m  RevolutionExtent=Custom  RevolutionAngle=mark_angle  RevolutionAngleUnits=deg  ExportConvexHullGeometry=off  InertiaType=CalculateFromGeometry  BasedOnType=Density  Density=1e-3  DensityUnits=kg/(m^3)  Mass=1  MassUnits=kg  CenterOfMass=[0 0 0]  CenterOfMassUnits=m  MomentsOfInertia=[1 1 1]  MomentsOfInertiaUnits=kg*m^2  ProductsOfInertia=[0 0 0]  ProductsOfInertiaUnits=kg*m^2  GraphicType=FromGeometry  MarkerShape=Sphere  MarkerSize=10  GraphicVisPropType=SimpleVisualProperties  GraphicDiffuseColor=[0.4 0.0 0.4]  GraphicOpacity=mark_opacity  GraphicSpecularColor=[0.5 0.5 0.5 1.0]  GraphicAmbientColor=[0.15 0.15 0.15 1.0]  GraphicEmissiveColor=[0.0 0.0 0.0 1.0]  GraphicShininess=75  DoExposeReferenceFrame=on  SerializedFrames=<Frames/>
  Vis2 : sm_lib/Body Elements/Revolved Solid  RevolutionCrossSection=[outer_rad*mark_radius(1) ring_length/2*1.002; inner_rad*mark_radius(2) ring_length/2*1.002; inner_rad*mark_radius(2) -ring_length/2*1.002; outer_rad*mark_radius(1) -ring_length/2*1.002]  RevolutionCrossSectionUnits=m  RevolutionExtent=Custom  RevolutionAngle=mark_angle  RevolutionAngleUnits=deg  ExportConvexHullGeometry=off  InertiaType=CalculateFromGeometry  BasedOnType=Density  Density=1e-3  DensityUnits=kg/(m^3)  Mass=1  MassUnits=kg  CenterOfMass=[0 0 0]  CenterOfMassUnits=m  MomentsOfInertia=[1 1 1]  MomentsOfInertiaUnits=kg*m^2  ProductsOfInertia=[0 0 0]  ProductsOfInertiaUnits=kg*m^2  GraphicType=FromGeometry  MarkerShape=Sphere  MarkerSize=10  GraphicVisPropType=SimpleVisualProperties  GraphicDiffuseColor=[0.4 0.0 0.4]  GraphicOpacity=mark_opacity  GraphicSpecularColor=[0.5 0.5 0.5 1.0]  GraphicAmbientColor=[0.15 0.15 0.15 1.0]  GraphicEmissiveColor=[0.0 0.0 0.0 1.0]  GraphicShininess=75  DoExposeReferenceFrame=on  SerializedFrames=<Frames/>
  R : PMIOPort  Side=Left
  connections:
  R/RConn1 -- Ring/RConn1 -- Transform Vis2/LConn1 -- Vis1/RConn1
  Vis2/RConn1 -- Transform Vis2/RConn1

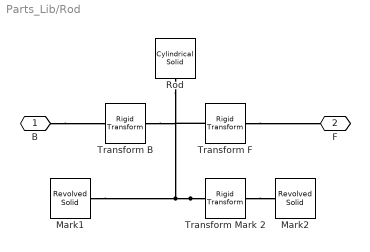
== system Parts_Lib/Rod ==
  Mark1 : sm_lib/Body Elements/Revolved Solid  RevolutionCrossSection=mark_xsec  RevolutionCrossSectionUnits=m  RevolutionExtent=Custom  RevolutionAngle=mark_angle_range  RevolutionAngleUnits=deg  ExportConvexHullGeometry=off  InertiaType=CalculateFromGeometry  BasedOnType=Density  Density=0  DensityUnits=kg/m^3  Mass=1  MassUnits=kg  CenterOfMass=[0 0 0]  CenterOfMassUnits=m  MomentsOfInertia=[1 1 1]  MomentsOfInertiaUnits=kg*m^2  ProductsOfInertia=[1 1 1]  ProductsOfInertiaUnits=kg*m^2  GraphicType=FromGeometry  MarkerShape=Sphere  MarkerSize=10  GraphicVisPropType=SimpleVisualProperties  GraphicDiffuseColor=mark_color  GraphicOpacity=mark_1_opc  GraphicSpecularColor=[0.5 0.5 0.5 1.0]  GraphicAmbientColor=[0.15 0.15 0.15 1.0]  GraphicEmissiveColor=[0.0 0.0 0.0 1.0]  GraphicShininess=75  DoExposeReferenceFrame=on  SerializedFrames=<Frames/>
  Mark2 : sm_lib/Body Elements/Revolved Solid  RevolutionCrossSection=mark_xsec  RevolutionCrossSectionUnits=m  RevolutionExtent=Custom  RevolutionAngle=mark_angle_range  RevolutionAngleUnits=deg  ExportConvexHullGeometry=off  InertiaType=CalculateFromGeometry  BasedOnType=Density  Density=0  DensityUnits=kg/m^3  Mass=1  MassUnits=kg  CenterOfMass=[0 0 0]  CenterOfMassUnits=m  MomentsOfInertia=[1 1 1]  MomentsOfInertiaUnits=kg*m^2  ProductsOfInertia=[1 1 1]  ProductsOfInertiaUnits=kg*m^2  GraphicType=FromGeometry  MarkerShape=Sphere  MarkerSize=10  GraphicVisPropType=SimpleVisualProperties  GraphicDiffuseColor=mark_color  GraphicOpacity=mark_2_opc  GraphicSpecularColor=[0.5 0.5 0.5 1.0]  GraphicAmbientColor=[0.15 0.15 0.15 1.0]  GraphicEmissiveColor=[0.0 0.0 0.0 1.0]  GraphicShininess=75  DoExposeReferenceFrame=on  SerializedFrames=<Frames/>
  Rod : sm_lib/Body Elements/Cylindrical Solid  CylinderRadius=rod_rad  CylinderRadiusUnits=m  CylinderLength=rod_len  CylinderLengthUnits=m  ExportEntireGeometry=off  InertiaType=CalculateFromGeometry  BasedOnType=Density  Density=rod_rho  DensityUnits=kg/(m^3)  Mass=1  MassUnits=kg  CenterOfMass=[0 0 0]  CenterOfMassUnits=m  MomentsOfInertia=[1 1 1]  MomentsOfInertiaUnits=kg*m^2  ProductsOfInertia=[0 0 0]  ProductsOfInertiaUnits=kg*m^2  GraphicType=FromGeometry  MarkerShape=Sphere  MarkerSize=10  GraphicVisPropType=SimpleVisualProperties  GraphicDiffuseColor=rod_color  GraphicOpacity=1.0  GraphicSpecularColor=[0.5 0.5 0.5 1.0]  GraphicAmbientColor=[0.15 0.15 0.15 1.0]  GraphicEmissiveColor=[0.0 0.0 0.0 1.0]  GraphicShininess=75  DoExposeReferenceFrame=on  SerializedFrames=<Frames/>
  Transform Mark 2 : sm_lib/Frames and Transforms/Rigid Transform  RotationMethod=StandardAxis  FollAlignAxisA=+X  BaseAlignAxisA=+Y  FollAlignAxisB=+Y  BaseAlignAxisB=+Z  RotationStandardAxis=+Z  RotationAngle=180  RotationAngleUnits=deg  RotationArbitraryAxis=[0 0 1]  RotationSequenceAxes=FollowerAxes  RotationSequence=XYX  RotationSequenceAngles=[0 0 0]  RotationSequenceAnglesUnits=deg  RotationMatrix=[1 0 0; 0 1 0; 0 0 1]  Quaternion=[1 0 0 0]  TranslationMethod=None  TranslationCartesianOffset=[0 0 0]  TranslationCartesianOffsetUnits=m  TranslationStandardAxis=+Z  TranslationStandardOffset=0  TranslationStandardOffsetUnits=m  TranslationROffset=0  TranslationROffsetUnits=m  TranslationThetaOffset=0  TranslationThetaOffsetUnits=deg  TranslationZOffset=0  TranslationZOffsetUnits=m
  Transform B : sm_lib/Frames and Transforms/Rigid Transform  RotationMethod=None  FollAlignAxisA=+X  BaseAlignAxisA=+Y  FollAlignAxisB=+Y  BaseAlignAxisB=+Z  RotationStandardAxis=+Z  RotationAngle=0.0  RotationAngleUnits=deg  RotationArbitraryAxis=[0 0 1]  RotationSequenceAxes=FollowerAxes  RotationSequence=XYX  RotationSequenceAngles=[0 0 0]  RotationSequenceAnglesUnits=deg  RotationMatrix=[1 0 0; 0 1 0; 0 0 1]  Quaternion=[1 0 0 0]  TranslationMethod=StandardAxis  TranslationCartesianOffset=[0 0 0]  TranslationCartesianOffsetUnits=m  TranslationStandardAxis=+Z  TranslationStandardOffset=rod_len/2*z_ori  TranslationStandardOffsetUnits=m  TranslationROffset=0  TranslationROffsetUnits=m  TranslationThetaOffset=0  TranslationThetaOffsetUnits=deg  TranslationZOffset=0  TranslationZOffsetUnits=m
  Transform F : sm_lib/Frames and Transforms/Rigid Transform  RotationMethod=None  FollAlignAxisA=+X  BaseAlignAxisA=+Y  FollAlignAxisB=+Y  BaseAlignAxisB=+Z  RotationStandardAxis=+Z  RotationAngle=0.0  RotationAngleUnits=deg  RotationArbitraryAxis=[0 0 1]  RotationSequenceAxes=FollowerAxes  RotationSequence=XYX  RotationSequenceAngles=[0 0 0]  RotationSequenceAnglesUnits=deg  RotationMatrix=[1 0 0; 0 1 0; 0 0 1]  Quaternion=[1 0 0 0]  TranslationMethod=StandardAxis  TranslationCartesianOffset=[0 0 0]  TranslationCartesianOffsetUnits=m  TranslationStandardAxis=+Z  TranslationStandardOffset=rod_len/2*z_ori  TranslationStandardOffsetUnits=m  TranslationROffset=0  TranslationROffsetUnits=m  TranslationThetaOffset=0  TranslationThetaOffsetUnits=deg  TranslationZOffset=0  TranslationZOffsetUnits=m
  B : PMIOPort  Side=Left
  F : PMIOPort  Port=2  Side=Right
  connections:
  Transform F/RConn1 -- F/RConn1
  B/RConn1 -- Transform B/LConn1
  Transform Mark 2/RConn1 -- Mark2/RConn1
  Transform Mark 2/LConn1 -- Mark1/RConn1 -- Transform F/LConn1 -- Transform B/RConn1 -- Rod/RConn1

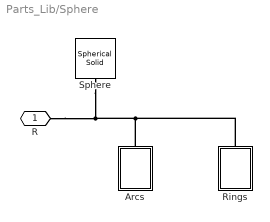
== system Parts_Lib/Sphere ==
  Arcs : Subsystem
  Rings : Subsystem
  Sphere : sm_lib/Body Elements/Spherical Solid  SphereRadius=sph_radius  SphereRadiusUnits=m  ExportEntireGeometry=off  InertiaType=CalculateFromGeometry  BasedOnType=Density  Density=sph_density  DensityUnits=kg/(m^3)  Mass=30e-3  MassUnits=kg  CenterOfMass=[0 0 0]  CenterOfMassUnits=m  MomentsOfInertia=[1 1 1]*1.358e-6  MomentsOfInertiaUnits=kg*m^2  ProductsOfInertia=[0 0 0]  ProductsOfInertiaUnits=kg*m^2  GraphicType=FromGeometry  MarkerShape=Sphere  MarkerSize=10  GraphicVisPropType=SimpleVisualProperties  GraphicDiffuseColor=[0.0 0.5 0.7]  GraphicOpacity=sph_opacity  GraphicSpecularColor=[0.5 0.5 0.5 1.0]  GraphicAmbientColor=[0.15 0.15 0.15 1.0]  GraphicEmissiveColor=[0.0 0.0 0.0 1.0]  GraphicShininess=75  DoExposeReferenceFrame=on  SerializedFrames=<Frames/>
  R : PMIOPort  Side=Left
  connections:
  R/RConn1 -- Rings/LConn1 -- Arcs/LConn1 -- Sphere/RConn1

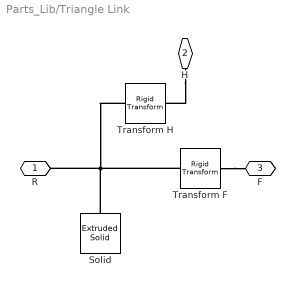
== system Parts_Lib/Triangle Link ==
  Solid : sm_lib/Body Elements/Extruded Solid  ExtrusionType=General  PolygonNumSides=3  PolygonOuterRadius=1  PolygonOuterRadiusUnits=m  ExportEntireGeometry=off  ExtrusionCrossSection=link_xsec  ExtrusionCrossSectionUnits=m  ExportConvexHullGeometry=off  ExtrusionLength=link_thickness  ExtrusionLengthUnits=m  InertiaType=CalculateFromGeometry  BasedOnType=Density  Density=link_rho  DensityUnits=kg/(m^3)  Mass=1  MassUnits=kg  CenterOfMass=[0 0 0]  CenterOfMassUnits=m  MomentsOfInertia=[1 1 1]  MomentsOfInertiaUnits=kg*m^2  ProductsOfInertia=[0 0 0]  ProductsOfInertiaUnits=kg*m^2  GraphicType=FromGeometry  MarkerShape=Sphere  MarkerSize=10  GraphicVisPropType=SimpleVisualProperties  GraphicDiffuseColor=link_color  GraphicOpacity=link_opc  GraphicSpecularColor=[0.5 0.5 0.5 1.0]  GraphicAmbientColor=[0.15 0.15 0.15 1.0]  GraphicEmissiveColor=[0.0 0.0 0.0 1.0]  GraphicShininess=75  DoExposeReferenceFrame=on  SerializedFrames=<Frames/>
  Transform F : sm_lib/Frames and Transforms/Rigid Transform  RotationMethod=None  FollAlignAxisA=+X  BaseAlignAxisA=+Y  FollAlignAxisB=+Y  BaseAlignAxisB=+Z  RotationStandardAxis=+Z  RotationAngle=0.0  RotationAngleUnits=deg  RotationArbitraryAxis=[0 0 1]  RotationSequenceAxes=FollowerAxes  RotationSequence=XYX  RotationSequenceAngles=[0 0 0]  RotationSequenceAnglesUnits=deg  RotationMatrix=[1 0 0; 0 1 0; 0 0 1]  Quaternion=[1 0 0 0]  TranslationMethod=StandardAxis  TranslationCartesianOffset=[0 0 0]  TranslationCartesianOffsetUnits=m  TranslationStandardAxis=+X  TranslationStandardOffset=link_len  TranslationStandardOffsetUnits=m  TranslationROffset=0  TranslationROffsetUnits=m  TranslationThetaOffset=0  TranslationThetaOffsetUnits=deg  TranslationZOffset=0  TranslationZOffsetUnits=m
  Transform H : sm_lib/Frames and Transforms/Rigid Transform  RotationMethod=None  FollAlignAxisA=+X  BaseAlignAxisA=+Y  FollAlignAxisB=+Y  BaseAlignAxisB=+Z  RotationStandardAxis=+Z  RotationAngle=0.0  RotationAngleUnits=deg  RotationArbitraryAxis=[0 0 1]  RotationSequenceAxes=FollowerAxes  RotationSequence=XYX  RotationSequenceAngles=[0 0 0]  RotationSequenceAnglesUnits=deg  RotationMatrix=[1 0 0; 0 1 0; 0 0 1]  Quaternion=[1 0 0 0]  TranslationMethod=Cartesian  TranslationCartesianOffset=[link_xlen*link_len link_height 0]  TranslationCartesianOffsetUnits=m  TranslationStandardAxis=+X  TranslationStandardOffset=0  TranslationStandardOffsetUnits=m  TranslationROffset=0  TranslationROffsetUnits=m  TranslationThetaOffset=0  TranslationThetaOffsetUnits=deg  TranslationZOffset=0  TranslationZOffsetUnits=m
  R : PMIOPort  Side=Left
  H : PMIOPort  Port=2  Side=Right
  F : PMIOPort  Port=3  Side=Right
  connections:
  H/RConn1 -- Transform H/RConn1
  Transform F/LConn1 -- Transform H/LConn1 -- Solid/RConn1 -- R/RConn1
  Transform F/RConn1 -- F/RConn1
